simulink model "enr312_temperature"  (R2026a)
settings: Solver=ode45  StopTime=Tend  MaxStep=0.01  RelTol=1e-6
model workspace (MAT data in the model file):
  Cth = 150
  Kd = 0
  Ki = 0
  Kp = 50
  N = 10
  Pbulb = 60
  Rth = 1
  SP = 45
  Ta = 30
  Tend = 900
  Ts = 0.01
  ambStep = 0
  delay = 3
  eta = 0.9
  hyst = 1
  modeSel = 1
  olPct = 100
  perDHT = 1
  resDHT = 1
  tAmb = 1000000000
  tauS = 10
  uTop = 255
libraries: slpidlib x1
settings Model: Creator=odyssix  LastModifiedBy=odyssix

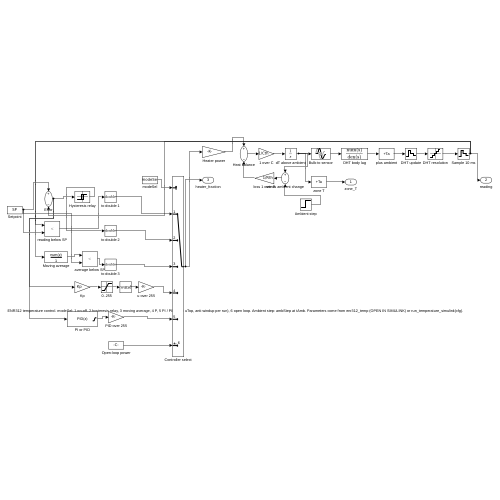
[thumbnail: Simulink's stored preview of the top-level diagram]
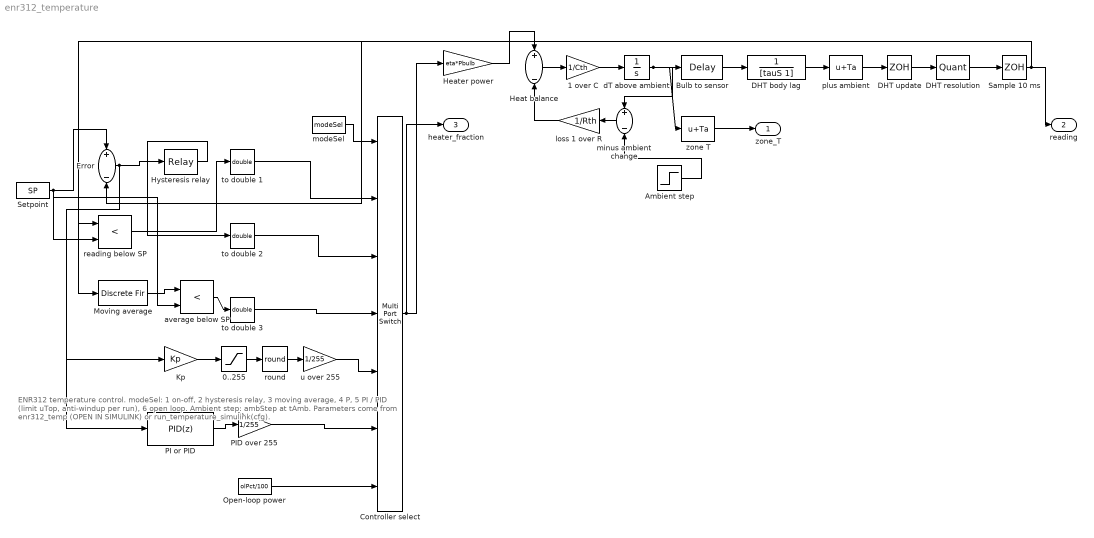
== system enr312_temperature ==
  note: ENR312 temperature control. modeSel: 1 on-off, 2 hysteresis relay, 3 moving average, 4 P, 5 PI / PID (limit uTop, anti-windup per run), 6 open loop. Ambient step: ambStep at tAmb. Parameters come from enr312_temp (OPEN IN SIMULINK) or run_temperature_simulink(cfg).
  0..255 : Saturate  UpperLimit=uTop  LowerLimit=0
  1 over C : Gain  Gain=1/Cth
  Ambient step : Step  Time=tAmb  FinalValue=ambStep  SampleTime=0
  Bulb to sensor : TransportDelay  DelayTime=delay  BufferSize=4096
  Controller select : MultiPortSwitch  Inputs=6  SaturateOnIntegerOverflow=off  InputSameDT=off
  DHT body lag : TransferFcn  Denominator=[tauS 1]
  DHT resolution : Quantizer  QuantizationInterval=resDHT
  DHT update : ZeroOrderHold  SampleTime=perDHT
  Error : Sum  Inputs=+-
  Heat balance : Sum  Inputs=+-
  Heater power : Gain  Gain=eta*Pbulb
  Hysteresis relay : Relay  OnSwitchValue=hyst/2  OffSwitchValue=-hyst/2
  Kp : Gain  Gain=Kp
  Moving average : DiscreteFir  Coefficients=ones(1,N)/N  SampleTime=Ts
  Open-loop power : Constant  Value=olPct/100
  PI or PID : slpidlib/PID Controller  Controller=PID  Form=Parallel  TimeDomain=Discrete-time  UseExternalTs=off  SampleTime=Ts  IntegratorMethod=Forward Euler  FilterMethod=Backward Euler  ControllerParametersSource=internal  P=Kp  I=Ki  UseKiTs=off  D=Kd  UseExternalDerivativeSource=off  N=1  UseFilter=on  TunerSelectOption=Transfer Function Based (PID Tuner App)  InitialConditionSource=internal  InitialConditionForIntegrator=0  InitialConditionForFilter=0  DifferentiatorICPrevScaledInput=0  ExternalReset=none  TrackingMode=off  Kt=1  LimitOutput=on  SatLimitsSource=internal  UpperSaturationLimit=uTop  LowerSaturationLimit=0  LinearizeAsGain=off  AntiWindupMode=clamping  Kb=1  LimitIntegrator=off  UpperIntegratorSaturationLimit=inf  LowerIntegratorSaturationLimit=-inf  POutMin=[]  POutMax=[]  IOutMin=[]  IOutMax=[]  DOutMin=[]  DOutMax=[]  NOutMin=[]  NOutMax=[]  SumOutMin=[]  SumOutMax=[]  SaturationOutMin=[]  SaturationOutMax=[]  PParamMin=[]  PParamMax=[]  IParamMin=[]  IParamMax=[]  DParamMin=[]  DParamMax=[]  NParamMin=[]  NParamMax=[]  KbParamMin=[]  KbParamMax=[]  KtParamMin=[]  KtParamMax=[]  KbOutMin=[]  KbOutMax=[]  KtOutMin=[]  KtOutMax=[]  IntegratorOutMin=[]  IntegratorOutMax=[]  FilterOutMin=[]  FilterOutMax=[]  SumI1OutMin=[]  SumI1OutMax=[]  SumI2OutMin=[]  SumI2OutMax=[]  SumI3OutMin=[]  SumI3OutMax=[]  SumI4OutMin=[]  SumI4OutMax=[]  SumDOutMin=[]  SumDOutMax=[]  DifferentiatorOutMin=[]  DifferentiatorOutMax=[]  FilterDiffOutCoefMin=[]  FilterDiffOutCoefMax=[]  ReciprocalOutMin=[]  ReciprocalOutMax=[]  SumDenOutMin=[]  SumDenOutMax=[]  SumNumOutMin=[]  SumNumOutMax=[]  DivideOutMin=[]  DivideOutMax=[]  UdiffTsProdOutMin=[]  UdiffTsProdOutMax=[]  NTsProdOutMin=[]  NTsProdOutMax=[]  UintegralTsProdOutMin=[]  UintegralTsProdOutMax=[]  UngainTsProdOutMin=[]  UngainTsProdOutMax=[]  ClampingZeroOutDataTypeStr=Inherit: Inherit via back propagation  ClampingZeroOutMin=[]  ClampingZeroOutMax=[]  FilterDenConstantOutDataTypeStr=Inherit: Inherit via back propagation  FilterDenConstantOutMin=[]  FilterDenConstantOutMax=[]  PCopyOutDataTypeStr=Inherit: Inherit via back propagation  PCopyOutMin=[]  PCopyOutMax=[]  NCopyOutDataTypeStr=Inherit: Inherit via back propagation  NCopyOutMin=[]  NCopyOutMax=[]  IntegratorContinuousStateAttributes=''  IntegratorStateMustResolveToSignalObject=off  IntegratorRTWStateStorageClass=Auto  FilterContinuousStateAttributes=''  FilterStateMustResolveToSignalObject=off  FilterRTWStateStorageClass=Auto  ParallelPVariant=InternalParameters  IdealPVariant=Disabled  IVariant=InternalParameters  DVariant=InternalParameters  IntegratorVariant=Discrete  SatVariant=Enabled  AWVariant=DiscClampingParallel  PCopyVariant=Disabled  TRVariant=Disabled  FdbkBlocksVariant=Forward  IdealPFdbkVariant=Disabled  SatFdbkVariant=Disabled  DerivativeFilterVariant=BackwardEulerFilter  NVariant=InternalParameters  NCopyVariant=InternalParameters  FilterICVariant=InternalICsFilter  IntegratorICVariant=InternalICs  ExternalResetVariant=Disabled  TRSumVariant=Passthrough  SumFdbkVariant=Disabled  SumVariant=Sum_PID  TsampFilterVariant=InternalTs  TsampNgainVariant=Passthrough  TsampIntegralVariant=Disabled_SignalSpec  ExternalSaturationOutDataTypeStr=Inherit: Same as second input  DerivativeSourceVariant=ErrorSignal  PreIntVariant=InternalPreInt
      settings: LibrarySourceBlock=simulink/Discrete/Discrete PID Controller
  PID over 255 : Gain  Gain=1/255
  Sample 10 ms : ZeroOrderHold  SampleTime=Ts
  Setpoint : Constant  Value=SP
  average below SP : RelationalOperator  Operator=<  OutDataTypeStr=boolean  RndMeth=Simplest  InputSameDT=off
  dT above ambient : Integrator
  loss 1 over R : Gain  Gain=1/Rth
  minus ambient change : Sum  Inputs=+-
  modeSel : Constant  Value=modeSel
  plus ambient : Bias  Bias=Ta  SaturateOnIntegerOverflow=off
  reading below SP : RelationalOperator  Operator=<  OutDataTypeStr=boolean  RndMeth=Simplest  InputSameDT=off
  round : Rounding  Operator=round
  to double 1 : DataTypeConversion  OutDataTypeStr=double  SaturateOnIntegerOverflow=off  RndMeth=Floor
  to double 2 : DataTypeConversion  OutDataTypeStr=double  SaturateOnIntegerOverflow=off  RndMeth=Floor
  to double 3 : DataTypeConversion  OutDataTypeStr=double  SaturateOnIntegerOverflow=off  RndMeth=Floor
  u over 255 : Gain  Gain=1/255
  zone T : Bias  Bias=Ta  SaturateOnIntegerOverflow=off
  zone_T : Outport
  reading : Outport  Port=2
  heater_fraction : Outport  Port=3
  wires:
  Heater power/1 -> Heat balance/1
  Heat balance/1 -> 1 over C/1
  1 over C/1 -> dT above ambient/1
  dT above ambient/1 -> minus ambient change/1, Bulb to sensor/1, zone T/1
  Ambient step/1 -> minus ambient change/2
  minus ambient change/1 -> loss 1 over R/1
  loss 1 over R/1 -> Heat balance/2
  Bulb to sensor/1 -> DHT body lag/1
  DHT body lag/1 -> plus ambient/1
  plus ambient/1 -> DHT update/1
  DHT update/1 -> DHT resolution/1
  DHT resolution/1 -> Sample 10 ms/1
  zone T/1 -> zone_T/1
  Sample 10 ms/1 -> reading/1, Error/2, reading below SP/1, Moving average/1
  Setpoint/1 -> Error/1, reading below SP/2, average below SP/2
  Error/1 -> Hysteresis relay/1, Kp/1, PI or PID/1
  Moving average/1 -> average below SP/1
  Kp/1 -> 0..255/1
  0..255/1 -> round/1
  round/1 -> u over 255/1
  reading below SP/1 -> to double 1/1
  Hysteresis relay/1 -> to double 2/1
  average below SP/1 -> to double 3/1
  modeSel/1 -> Controller select/1
  to double 1/1 -> Controller select/2
  to double 2/1 -> Controller select/3
  to double 3/1 -> Controller select/4
  u over 255/1 -> Controller select/5
  PI or PID/1 -> PID over 255/1
  PID over 255/1 -> Controller select/6
  Open-loop power/1 -> Controller select/7
  Controller select/1 -> Heater power/1, heater_fraction/1
